simulink model "ConfiguredHevMmVirtualVehicle"  (R2025b)
settings: configuration reference "VehicleVariable" (kept outside this file)
StartFcn:
  | %tic
StopFcn:
  | %toc
model workspace (MAT data in the model file):
  ExtDrvCmdsSwitch : Simulink.Parameter (value not decoded)
  ExtDrvRefSwitch : Simulink.Parameter (value not decoded)
  ExtEnvSwitch : Simulink.Parameter (value not decoded)
  ExtGndSwitch : Simulink.Parameter (value not decoded)
symbols that are objects in the model workspace (value not decoded): ExtDrvCmdsSwitch, ExtDrvRefSwitch, ExtEnvSwitch, ExtGndSwitch
undefined symbols (not defined in the file or in its folder): AmbTemp, BaroPress, CurvGradRef, CurvRef, DCM, DriverAeroRes, DriverDrivelineRes, DriverInitialGear, DriverPreviewDist, DriverRollRes, DriverShiftTime, DriverTimeConst, DriverTractiveForce, EnvAbsPrs, EnvAirTemp, EnvGrvty, EnvNomFrictionScaling, EnvNominalGrade, EnvScnFrictionMap, EnvScnFrictionMapXBpts, EnvScnFrictionMapYBpts, EnvScnHeightMap, EnvScnHeightMapXBpts, EnvScnHeightMapYBpts, EnvWindVelX, EnvWindVelY, EnvWindVelZ, Gnd, Grade, HazzardCmd, HighBeamCmd, lambda_mux, LeftSignalCmd, LngRef, LowBeamCmd, LtrRef, PhiRef, PlntVehDstCGFrntAxl, PlntVehDstCGRearAxl, PlntVehInitLatPos, PlntVehInitLongPos, PlntVehInitPitchAng, PlntVehInitRollAng, PlntVehInitVertPos, PlntVehInitYawAng, PlntVehMass, PlntVehTrckWdth, PlntVehYawMomentInertia, PlntWhlLdRadiusFrnt, PlntWhlLdRadiusRear, RightSignalCmd, ScnCRRadius, Sim3dSensor, Wind, XRef, YRef, Z
libraries: simulink x28, autolibutils x8, autolibsharedcommon x7, vehdynlibscenariocommon x7, vehdynlibviscommon x4, vehdynlibdriver x2, sim3dgroundtruthsensorlib x2, sim3dlib x2, autolibshared x2, sim3dautolib x2, sl3dlib x1, sharedtransform x1
(part 6 of 6)

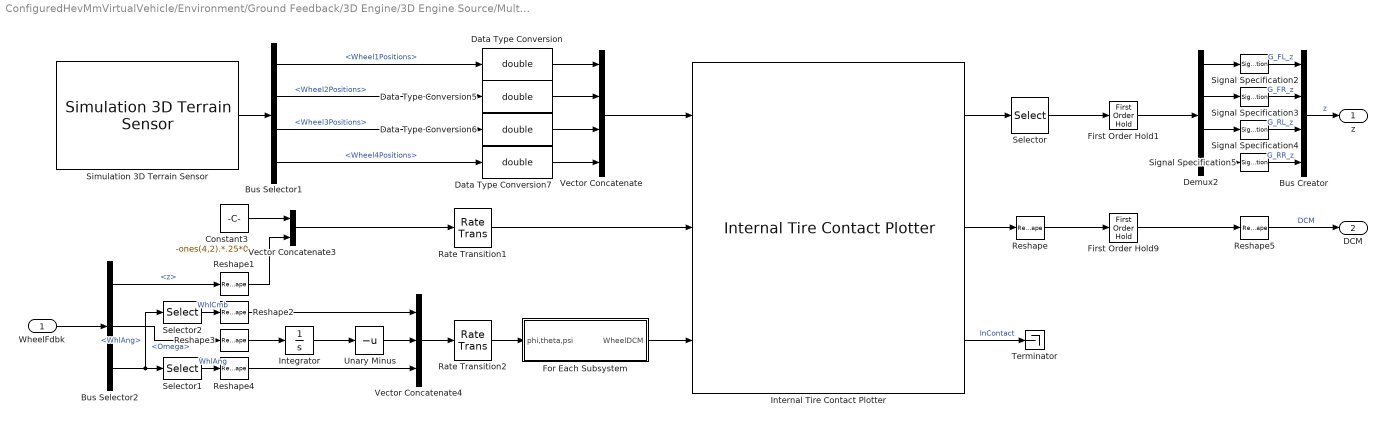
== system ConfiguredHevMmVirtualVehicle/Environment/Ground Feedback/3D Engine/3D Engine Source/Multiple Points ==
  WheelFdbk : Inport
  Bus Creator : BusCreator  Inputs=4
  Bus Selector1 : BusSelector  OutputSignals=Wheel1Positions,Wheel2Positions,Wheel3Positions,Wheel4Positions
  Bus Selector2 : BusSelector  OutputSignals=z,Omega,WhlAng
  Constant3 : Constant  Value=-ones(4,2).*.25*0
  Data Type Conversion{,5..7} (4 alike) : DataTypeConversion  OutDataTypeStr=double  SaturateOnIntegerOverflow=off  RndMeth=Floor
  Demux2 : Demux
  First Order Hold1 : FirstOrderHold  OutputAlgorithm=Fast (Minimize Error)  ErrorTolerance=.001
  First Order Hold9 : FirstOrderHold  InitialOutput=reshape(repmat(eye(3),1,1,4),[],1)  OutputAlgorithm=Fast (Minimize Error)  ErrorTolerance=.001
  For Each Subsystem : Subsystem  TreatAsAtomicUnit=on
  Integrator : Integrator  WrapState=on  ZeroCross=off
  Internal Tire Contact Plotter : vehdynlibviscommon/Internal Tire Contact Plotter  dispFig=off  numAxles=2  numWheelsPerAxle=2  wheelRad=.33  wheelWidth=.235  rayOrigins=[0.5 -0.5 0;0.4 -0.5 0;0.3 -0.5 0;0.19999999999999996 -0.5 0;0.099999999999999978 -0.5 0;0 -0.5 0;-0.099999999999999978 -0.5 0;-0.19999999999999996 -0.5 0;-0.3 -0.5 0;-0.4 -0.5 0;-0.5 -0.5 0;0.5 -0.4 0;0.4 -0.4 0;0.3 -0.4 0;0.19999999999999996 -0.4 0;0.099999999999999978 -0.4 0;0 -0.4 0;-0.099999999999999978 -0.4 0;-0.19999999999999996 -0.4 0;-0.3 -0.4 0;-0.4 -0.4 0;-0.5 -0.4 0;0.5 -0.3 0;0.4 -0.3 0;0.3 -0.3 0;0.19999999999999996 -0.3 0;0.099999999999999978 -0.3 0;0 -0.3 0;-0.099999999999999978 -0.3 0;-0.19999999999999996 -0.3 0;-0.3 -0.3 0;-0.4 -0.3 0;-0.5 -0.3 0;0.5 -0.19999999999999996 0;0.4 -0.19999999999999996 0;0.3 -0.19999999999999996 0;0.19999999999999996 -0.19999999999999996 0;0.099999999999999978 -0.19999999999999996 0;0 -0.19999999999999996 0;-0.099999999999999978 -0.19999999999999996 0;-0.19999999999999996 -0.19999999999999996 0;-0.3 -0.19999999999999996 0;-0.4 -0.19999999999999996 0;-0.5 -0.19999999999999996 0;0.5 -0.099999999999999978 0;0.4 -0.099999999999999978 0;0.3 -0.099999999999999978 0;0.19999999999999996 -0.099999999999999978 0;0.099999999999999978 -0.099999999999999978 0;0 -0.099999999999999978 0;-0.099999999999999978 -0.099999999999999978 0;-0.19999999999999996 -0.099999999999999978 0;-0.3 -0.099999999999999978 0;-0.4 -0.099999999999999978 0;-0.5 -0.099999999999999978 0;0.5 0 0;0.4 0 0;0.3 0 0;0.19999999999999996 0 0;0.099999999999999978 0 0;0 0 0;-0.099999999999999978 0 0;-0.19999999999999996 0 0;-0.3 0 0;-0.4 0 0;-0.5 0 0;0.5 0.099999999999999978 0;0.4 0.099999999999999978 0;0.3 0.099999999999999978 0;0.19999999999999996 0.099999999999999978 0;0.099999999999999978 0.099999999999999978 0;0 0.099999999999999978 0;-0.099999999999999978 0.099999999999999978 0;-0.19999999999999996 0.099999999999999978 0;-0.3 0.099999999999999978 0;-0.4 0.099999999999999978 0;-0.5 0.099999999999999978 0;0.5 0.19999999999999996 0;0.4 0.19999999999999996 0;0.3 0.19999999999999996 0;0.19999999999999996 0.19999999999999996 0;0.099999999999999978 0.19999999999999996 0;0 0.19999999999999996 0;-0.099999999999999978 0.19999999999999996 0;-0.19999999999999996 0.19999999999999996 0;-0.3 0.19999999999999996 0;-0.4 0.19999999999999996 0;-0.5 0.19999999999999996 0;0.5 0.3 0;0.4 0.3 0;0.3 0.3 0;0.19999999999999996 0.3 0;0.099999999999999978 0.3 0;0 0.3 0;-0.099999999999999978 0.3 0;-0.19999999999999996 0.3 0;-0.3 0.3 0;-0.4 0.3 0;-0.5 0.3 0;0.5 0.4 0;0.4 0.4 0;0.3 0.4 0;0.19999999999999996 0.4 0;0.099999999999999978 0.4 0;0 0.4 0;-0.099999999999999978 0.4 0;-0.19999999999999996 0.4 0;-0.3 0.4 0;-0.4 0.4 0;-0.5 0.4 0;0.5 0.5 0;0.4 0.5 0;0.3 0.5 0;0.19999999999999996 0.5 0;0.099999999999999978 0.5 0;0 0.5 0;-0.099999999999999978 0.5 0;-0.19999999999999996 0.5 0;-0.3 0.5 0;-0.4 0.5 0;-0.5 0.5 0]
  Rate Transition1 : RateTransition  Integrity=off  Deterministic=off  OutPortSampleTime=.01
  Rate Transition2 : RateTransition  Integrity=off  Deterministic=off  OutPortSampleTime=.01
  Reshape : Reshape  OutputDimensionality=Column vector (2-D)
  Reshape1 : Reshape  OutputDimensionality=Column vector (2-D)
  Reshape2 : Reshape  OutputDimensionality=Row vector (2-D)
  Reshape3 : Reshape  OutputDimensionality=Row vector (2-D)
  Reshape4 : Reshape  OutputDimensionality=Row vector (2-D)
  Reshape5 : Reshape  OutputDimensionality=Customize  OutputDimensions=[3,3,4]
  Selector : Selector  NumberOfDimensions=2  InputPortWidth=3  IndexOptions=Select all,Index vector (dialog)  Indices=[1 3],3  OutputSizes=1,1
  Selector1 : Selector  NumberOfDimensions=2  InputPortWidth=3  IndexOptions=Index vector (dialog),Select all  Indices=[3],1  OutputSizes=1,1
  Selector2 : Selector  NumberOfDimensions=2  InputPortWidth=3  IndexOptions=Index vector (dialog),Select all  Indices=[1],1  OutputSizes=1,1
  Signal Specification{2..5} (4 alike) : SignalSpecification  Unit=m
  Simulation 3D Terrain Sensor : sim3dgroundtruthsensorlib/Simulation 3D Terrain Sensor  Priority=1  vehTagList={'Scene Origin';'SimulinkVehicle1';'0'}  sensorTag=Sim3dSensor�  sensorId=1  sensorName=Sim3dSensor�  vehTag=SimulinkVehicle1  CoordinateSystem=Default  tmountOffset=[0, 0, 0]  rmountOffset=[0,0,0,]  RayOrigins=[0.5 -0.5 0;0.4 -0.5 0;0.3 -0.5 0;0.19999999999999996 -0.5 0;0.099999999999999978 -0.5 0;0 -0.5 0;-0.099999999999999978 -0.5 0;-0.19999999999999996 -0.5 0;-0.3 -0.5 0;-0.4 -0.5 0;-0.5 -0.5 0;0.5 -0.4 0;0.4 -0.4 0;0.3 -0.4 0;0.19999999999999996 -0.4 0;0.099999999999999978 -0.4 0;0 -0.4 0;-0.099999999999999978 -0.4 0;-0.19999999999999996 -0.4 0;-0.3 -0.4 0;-0.4 -0.4 0;-0.5 -0.4 0;0.5 -0.3 0;0.4 -0.3 0;0.3 -0.3 0;0.19999999999999996 -0.3 0;0.099999999999999978 -0.3 0;0 -0.3 0;-0.099999999999999978 -0.3 0;-0.19999999999999996 -0.3 0;-0.3 -0.3 0;-0.4 -0.3 0;-0.5 -0.3 0;0.5 -0.19999999999999996 0;0.4 -0.19999999999999996 0;0.3 -0.19999999999999996 0;0.19999999999999996 -0.19999999999999996 0;0.099999999999999978 -0.19999999999999996 0;0 -0.19999999999999996 0;-0.099999999999999978 -0.19999999999999996 0;-0.19999999999999996 -0.19999999999999996 0;-0.3 -0.19999999999999996 0;-0.4 -0.19999999999999996 0;-0.5 -0.19999999999999996 0;0.5 -0.099999999999999978 0;0.4 -0.099999999999999978 0;0.3 -0.099999999999999978 0;0.19999999999999996 -0.099999999999999978 0;0.099999999999999978 -0.099999999999999978 0;0 -0.099999999999999978 0;-0.099999999999999978 -0.099999999999999978 0;-0.19999999999999996 -0.099999999999999978 0;-0.3 -0.099999999999999978 0;-0.4 -0.099999999999999978 0;-0.5 -0.099999999999999978 0;0.5 0 0;0.4 0 0;0.3 0 0;0.19999999999999996 0 0;0.099999999999999978 0 0;0 0 0;-0.099999999999999978 0 0;-0.19999999999999996 0 0;-0.3 0 0;-0.4 0 0;-0.5 0 0;0.5 0.099999999999999978 0;0.4 0.099999999999999978 0;0.3 0.099999999999999978 0;0.19999999999999996 0.099999999999999978 0;0.099999999999999978 0.099999999999999978 0;0 0.099999999999999978 0;-0.099999999999999978 0.099999999999999978 0;-0.19999999999999996 0.099999999999999978 0;-0.3 0.099999999999999978 0;-0.4 0.099999999999999978 0;-0.5 0.099999999999999978 0;0.5 0.19999999999999996 0;0.4 0.19999999999999996 0;0.3 0.19999999999999996 0;0.19999999999999996 0.19999999999999996 0;0.099999999999999978 0.19999999999999996 0;0 0.19999999999999996 0;-0.099999999999999978 0.19999999999999996 0;-0.19999999999999996 0.19999999999999996 0;-0.3 0.19999999999999996 0;-0.4 0.19999999999999996 0;-0.5 0.19999999999999996 0;0.5 0.3 0;0.4 0.3 0;0.3 0.3 0;0.19999999999999996 0.3 0;0.099999999999999978 0.3 0;0 0.3 0;-0.099999999999999978 0.3 0;-0.19999999999999996 0.3 0;-0.3 0.3 0;-0.4 0.3 0;-0.5 0.3 0;0.5 0.4 0;0.4 0.4 0;0.3 0.4 0;0.19999999999999996 0.4 0;0.099999999999999978 0.4 0;0 0.4 0;-0.099999999999999978 0.4 0;-0.19999999999999996 0.4 0;-0.3 0.4 0;-0.4 0.4 0;-0.5 0.4 0;0.5 0.5 0;0.4 0.5 0;0.3 0.5 0;0.19999999999999996 0.5 0;0.099999999999999978 0.5 0;0 0.5 0;-0.099999999999999978 0.5 0;-0.19999999999999996 0.5 0;-0.3 0.5 0;-0.4 0.5 0;-0.5 0.5 0]  RayDirections=[0 0 -1;0 0 -1;0 0 -1;0 0 -1;0 0 -1;0 0 -1;0 0 -1;0 0 -1;0 0 -1;0 0 -1;0 0 -1;0 0 -1;0 0 -1;0 0 -1;0 0 -1;0 0 -1;0 0 -1;0 0 -1;0 0 -1;0 0 -1;0 0 -1;0 0 -1;0 0 -1;0 0 -1;0 0 -1;0 0 -1;0 0 -1;0 0 -1;0 0 -1;0 0 -1;0 0 -1;0 0 -1;0 0 -1;0 0 -1;0 0 -1;0 0 -1;0 0 -1;0 0 -1;0 0 -1;0 0 -1;0 0 -1;0 0 -1;0 0 -1;0 0 -1;0 0 -1;0 0 -1;0 0 -1;0 0 -1;0 0 -1;0 0 -1;0 0 -1;0 0 -1;0 0 -1;0 0 -1;0 0 -1;0 0 -1;0 0 -1;0 0 -1;0 0 -1;0 0 -1;0 0 -1;0 0 -1;0 0 -1;0 0 -1;0 0 -1;0 0 -1;0 0 -1;0 0 -1;0 0 -1;0 0 -1;0 0 -1;0 0 -1;0 0 -1;0 0 -1;0 0 -1;0 0 -1;0 0 -1;0 0 -1;0 0 -1;0 0 -1;0 0 -1;0 0 -1;0 0 -1;0 0 -1;0 0 -1;0 0 -1;0 0 -1;0 0 -1;0 0 -1;0 0 -1;0 0 -1;0 0 -1;0 0 -1;0 0 -1;0 0 -1;0 0 -1;0 0 -1;0 0 -1;0 0 -1;0 0 -1;0 0 -1;0 0 -1;0 0 -1;0 0 -1;0 0 -1;0 0 -1;0 0 -1;0 0 -1;0 0 -1;0 0 -1;0 0 -1;0 0 -1;0 0 -1;0 0 -1;0 0 -1;0 0 -1;0 0 -1;0 0 -1;0 0 -1;0 0 -1;0 0 -1]  RayLengths=[20;20;20;20;20;20;20;20;20;20;20;20;20;20;20;20;20;20;20;20;20;20;20;20;20;20;20;20;20;20;20;20;20;20;20;20;20;20;20;20;20;20;20;20;20;20;20;20;20;20;20;20;20;20;20;20;20;20;20;20;20;20;20;20;20;20;20;20;20;20;20;20;20;20;20;20;20;20;20;20;20;20;20;20;20;20;20;20;20;20;20;20;20;20;20;20;20;20;20;20;20;20;20;20;20;20;20;20;20;20;20;20;20;20;20;20;20;20;20;20;20]  NumberOfWheels=4  VisualizeTraceLines=off  SampleTime=-1  aMode=2  ID=1
  Terminator : Terminator
  Unary Minus : UnaryMinus
  Vector Concatenate : Concatenate  NumInputs=4  Mode=Multidimensional array  ConcatenateDimension=3
  Vector Concatenate3 : Concatenate  Mode=Multidimensional array  ConcatenateDimension=2
  Vector Concatenate4 : Concatenate  NumInputs=3  Mode=Multidimensional array
  z : Outport
  DCM : Outport  Port=2
  wires:
  Data Type Conversion6/1 -> Vector Concatenate/3
  Selector/1 -> First Order Hold1/1
  Signal Specification5/1 -> Bus Creator/4  "G_RR_z"
  Bus Selector1/3 -> Data Type Conversion6/1  "<Wheel3Positions>"
  Demux2/2 -> Signal Specification3/1
  Data Type Conversion/1 -> Vector Concatenate/1
  Data Type Conversion5/1 -> Vector Concatenate/2
  Demux2/3 -> Signal Specification4/1
  Internal Tire Contact Plotter/1 -> Selector/1
  Internal Tire Contact Plotter/3 -> Terminator/1  "InContact"
  Vector Concatenate/1 -> Internal Tire Contact Plotter/1
  Data Type Conversion7/1 -> Vector Concatenate/4
  Bus Selector1/1 -> Data Type Conversion/1  "<Wheel1Positions>"
  Demux2/4 -> Signal Specification5/1
  Bus Creator/1 -> z/1  "z"
  Signal Specification2/1 -> Bus Creator/1  "G_FL_z"
  Bus Selector1/4 -> Data Type Conversion7/1  "<Wheel4Positions>"
  Signal Specification3/1 -> Bus Creator/2  "G_FR_z"
  Signal Specification4/1 -> Bus Creator/3  "G_RL_z"
  Bus Selector1/2 -> Data Type Conversion5/1  "<Wheel2Positions>"
  Demux2/1 -> Signal Specification2/1
  Simulation 3D Terrain Sensor/1 -> Bus Selector1/1
  Reshape5/1 -> DCM/1  "DCM"
  Internal Tire Contact Plotter/2 -> Reshape/1
  Integrator/1 -> Unary Minus/1
  Bus Selector2/2 -> Reshape3/1  "<Omega>"
  Vector Concatenate3/1 -> Rate Transition1/1
  For Each Subsystem/1(WheelDCM) -> Internal Tire Contact Plotter/3
  Reshape3/1 -> Integrator/1
  Vector Concatenate4/1 -> Rate Transition2/1
  Reshape4/1 -> Vector Concatenate4/3
  Rate Transition2/1 -> For Each Subsystem/1(phi,theta,psi)
  Reshape1/1 -> Vector Concatenate3/2
  WheelFdbk/1 -> Bus Selector2/1
  Bus Selector2/1 -> Reshape1/1  "<z>"
  Bus Selector2/3 -> Selector2/1, Selector1/1  "<WhlAng>"
  Constant3/1 -> Vector Concatenate3/1
  Reshape2/1 -> Vector Concatenate4/1
  Unary Minus/1 -> Vector Concatenate4/2
  Rate Transition1/1 -> Internal Tire Contact Plotter/2
  First Order Hold9/1 -> Reshape5/1
  Reshape/1 -> First Order Hold9/1
  First Order Hold1/1 -> Demux2/1
  Selector1/1 -> Reshape4/1  "WhlAng"
  Selector2/1 -> Reshape2/1  "WhlCmb"

== system ConfiguredHevMmVirtualVehicle/Environment/Ground Feedback/3D Engine/3D Engine Source/Single Point ==
  Bus Creator1 : BusCreator  Inputs=4
  Bus Selector2 : BusSelector  OutputSignals=Wheel1Positions,Wheel2Positions,Wheel3Positions,Wheel4Positions
  Constant2 : Constant  Value=repmat(eye(3),1,1,4)  SampleTime=-1
  Data Type Conversion{1..4} (4 alike) : DataTypeConversion  SaturateOnIntegerOverflow=off  RndMeth=Floor
  First Order Hold{5..8} (4 alike) : FirstOrderHold  ErrorTolerance=1
  Range Limiter{5..8} (4 alike) : Saturate  UpperLimit=1e3  LowerLimit=-1e3  ZeroCross=off
  Signal Specification{6..9} (4 alike) : SignalSpecification  Unit=m
  Simulation 3D Terrain Sensor1 : sim3dgroundtruthsensorlib/Simulation 3D Terrain Sensor  Priority=1  vehTagList={'Scene Origin';'SimulinkVehicle1'}  sensorTag=Sim3dSensor�  sensorId=1  sensorName=Sim3dSensor1  vehTag=SimulinkVehicle1  CoordinateSystem=Default  tmountOffset=[0, 0, 0]  rmountOffset=[0,0,0,]  RayOrigins=[0 0 1]  RayDirections=[0 0 -1]  RayLengths=20  NumberOfWheels=4  VisualizeTraceLines=off  SampleTime=-1  aMode=2  ID=1
  Zend Select{1..4} (4 alike) : Selector  NumberOfDimensions=2  InputPortWidth=3  IndexOptions=Select all,Index vector (dialog)  Indices=[1 3],3  OutputSizes=1,1
  z : Outport
  DCM : Outport  Port=2
  wires:
  Signal Specification6/1 -> Bus Creator1/1  "G_FL_z"
  Simulation 3D Terrain Sensor1/1 -> Bus Selector2/1
  Bus Selector2/4 -> Range Limiter8/1  "<Wheel4Positions>"
  Zend Select1/1 -> Data Type Conversion1/1
  Signal Specification7/1 -> Bus Creator1/2  "G_FR_z"
  Bus Selector2/2 -> Range Limiter6/1  "<Wheel2Positions>"
  Data Type Conversion3/1 -> First Order Hold7/1
  Data Type Conversion4/1 -> First Order Hold8/1
  Zend Select3/1 -> Data Type Conversion3/1
  First Order Hold6/1 -> Signal Specification7/1
  Zend Select2/1 -> Data Type Conversion2/1
  Data Type Conversion2/1 -> First Order Hold6/1
  Range Limiter6/1 -> Zend Select2/1
  Data Type Conversion1/1 -> First Order Hold5/1
  First Order Hold7/1 -> Signal Specification8/1
  Zend Select4/1 -> Data Type Conversion4/1
  Range Limiter8/1 -> Zend Select4/1
  Bus Selector2/1 -> Range Limiter5/1  "<Wheel1Positions>"
  First Order Hold8/1 -> Signal Specification9/1
  Bus Selector2/3 -> Range Limiter7/1  "<Wheel3Positions>"
  Range Limiter7/1 -> Zend Select3/1
  First Order Hold5/1 -> Signal Specification6/1
  Range Limiter5/1 -> Zend Select1/1
  Signal Specification8/1 -> Bus Creator1/3  "G_RL_z"
  Signal Specification9/1 -> Bus Creator1/4  "G_RR_z"
  Bus Creator1/1 -> z/1  "z"
  Constant2/1 -> DCM/1  "DCM"

== system ConfiguredHevMmVirtualVehicle/Environment/Ground Feedback/Ideal Inclined Plane/Ideal Inclined Plane/Enabled ==
  Z : Inport
  phi : Inport  Port=2
  theta : Inport  Port=3
  Disabled : Subsystem  VariantControl=plane3D==0
  Enabled : Subsystem  VariantControl=plane3D==1

== system ConfiguredHevMmVirtualVehicle/Environment/Subsystem/Estimated Grade/Variant Subsystem/Three-Axle ==
  Gnd : Inport
  Selector : Selector  InputPortWidth=6  IndexOptions=Index vector (dialog)  Indices=[1 2]  OutputSizes=1
  Selector1 : Selector  InputPortWidth=6  IndexOptions=Index vector (dialog)  Indices=[5 6]  OutputSizes=1
  F : Outport
  R : Outport  Port=2
  wires:
  Selector/1 -> F/1
  Gnd/1 -> Selector1/1, Selector/1
  Selector1/1 -> R/1

== system ConfiguredHevMmVirtualVehicle/Environment/Subsystem/Estimated Grade/Variant Subsystem/Two-Axle ==
  Gnd : Inport
  Selector : Selector  InputPortWidth=4  IndexOptions=Index vector (dialog)  Indices=[1 2]  OutputSizes=1
  Selector1 : Selector  InputPortWidth=4  IndexOptions=Index vector (dialog)  Indices=[3 4]  OutputSizes=1
  F : Outport
  R : Outport  Port=2
  wires:
  Selector1/1 -> R/1
  Selector/1 -> F/1
  Gnd/1 -> Selector1/1, Selector/1

== system ConfiguredHevMmVirtualVehicle/Environment/Varying Friction/Varying Friction/Road Track Friction/2D Lookup Tbl for Scaling Fctr (Lambda) ==
  XWhl : Inport  Partition=on  PartitionDimension=1  PartitionWidth=1  PartitionOffset=0
  YWhl : Inport  Port=2  Partition=on  PartitionDimension=1  PartitionWidth=1  PartitionOffset=0
  XBpt : Inport  Port=3
  YBpt : Inport  Port=4
  2-D Lookup Table : Lookup_n-D  BreakpointsForDimension1Source=Input port  BreakpointsForDimension1=xbr  BreakpointsForDimension2Source=Input port  BreakpointsForDimension2=ybr  Table=mutable  ExtrapMethod=Clip  InternalRulePriority=Speed  RndMeth=Simplest
      settings: InputPortMap=u0,u1,p5,p7
  For Each : ForEach  DisableCoverage=on
  Lambda for each whl : Outport  ConcatenationDimension=1
  wires:
  XWhl/1 -> 2-D Lookup Table/1
  YWhl/1 -> 2-D Lookup Table/2
  2-D Lookup Table/1 -> Lambda for each whl/1
  XBpt/1 -> 2-D Lookup Table/3
  YBpt/1 -> 2-D Lookup Table/4

== system ConfiguredHevMmVirtualVehicle/Environment/Varying Friction/Varying Friction/Road Track Friction/Creating Inertial Frm Bpt ==
  XCg : Inport
  YCg : Inport  Port=2
  Enable : EnablePort
  Add : Sum
  Add1 : Sum
  Constant1 : Constant  Value=ybr
  Constant3 : Constant  Value=xbr
  XBpt : Outport
  YBpt : Outport  Port=2
  wires:
  Add/1 -> XBpt/1
  Constant1/1 -> Add1/1
  Add1/1 -> YBpt/1
  Constant3/1 -> Add/2
  YCg/1 -> Add1/2
  XCg/1 -> Add/1

== system ConfiguredHevMmVirtualVehicle/Environment/Varying Friction/Varying Friction/Road Track Friction/En at t = 0 ==
  Clock1 : Clock
  Compare To Zero : simulink/Logic and Bit Operations/Compare To Zero  relop===  OutDataTypeStr=boolean
  Constant : Constant
  Constant2 : Constant  Value=0
  Switch1 : Switch  Criteria=u2 > Threshold  SaturateOnIntegerOverflow=off  InputSameDT=off
  Out1 : Outport
  wires:
  Clock1/1 -> Compare To Zero/1
  Constant2/1 -> Switch1/3
  Constant/1 -> Switch1/1
  Switch1/1 -> Out1/1
  Compare To Zero/1 -> Switch1/2

== system ConfiguredHevMmVirtualVehicle/Visualization/3D Engine/3D Engine/Scale/PartConcatenation ==
  BodyX : Inport
  BodyY : Inport  Port=2
  BodyZ : Inport  Port=3
  WheelFrontLeftX : Inport  Port=4
  WheelFrontLeftY : Inport  Port=5
  WheelFrontLeftZ : Inport  Port=6
  WheelFrontRightX : Inport  Port=7
  WheelFrontRightY : Inport  Port=8
  WheelFrontRightZ : Inport  Port=9
  WheelRearLeftX : Inport  Port=10
  WheelRearLeftY : Inport  Port=11
  WheelRearLeftZ : Inport  Port=12
  WheelRearRightX : Inport  Port=13
  WheelRearRightY : Inport  Port=14
  WheelRearRightZ : Inport  Port=15
  AllParts : Concatenate  NumInputs=5  Mode=Multidimensional array
  Body : Concatenate  NumInputs=3  Mode=Multidimensional array  ConcatenateDimension=2
  WheelFrontLeft : Concatenate  NumInputs=3  Mode=Multidimensional array  ConcatenateDimension=2
  WheelFrontRight : Concatenate  NumInputs=3  Mode=Multidimensional array  ConcatenateDimension=2
  WheelRearLeft : Concatenate  NumInputs=3  Mode=Multidimensional array  ConcatenateDimension=2
  WheelRearRight : Concatenate  NumInputs=3  Mode=Multidimensional array  ConcatenateDimension=2
  ConcatOut : Outport  VectorParamsAs1DForOutWhenUnconnected=off
  wires:
  WheelFrontRightZ/1 -> WheelFrontRight/3
  WheelRearLeftX/1 -> WheelRearLeft/1
  WheelRearRight/1 -> AllParts/5
  WheelRearLeftY/1 -> WheelRearLeft/2
  AllParts/1 -> ConcatOut/1
  WheelRearLeftZ/1 -> WheelRearLeft/3
  WheelRearRightY/1 -> WheelRearRight/2
  WheelFrontRightX/1 -> WheelFrontRight/1
  WheelFrontRightY/1 -> WheelFrontRight/2
  WheelRearRightZ/1 -> WheelRearRight/3
  WheelFrontRight/1 -> AllParts/3
  WheelRearLeft/1 -> AllParts/4
  Body/1 -> AllParts/1
  WheelRearRightX/1 -> WheelRearRight/1
  WheelFrontLeft/1 -> AllParts/2
  BodyY/1 -> Body/2
  WheelFrontLeftY/1 -> WheelFrontLeft/2
  WheelFrontLeftZ/1 -> WheelFrontLeft/3
  WheelFrontLeftX/1 -> WheelFrontLeft/1
  BodyZ/1 -> Body/3
  BodyX/1 -> Body/1

== system ConfiguredHevMmVirtualVehicle/Visualization/3D Engine/3D Engine/Trailer/No Trailer ==
  VehFdbk : Inport
  Terminator : Terminator
  wires:
  VehFdbk/1 -> Terminator/1

== system ConfiguredHevMmVirtualVehicle/Visualization/3D Engine/3D Engine/Trailer/One-Axle Trailer ==
  VehFdbk : Inport
  Simulation 3D Trailer : sim3dautolib/Simulation 3D Trailer  Priority=-1  Mesh=One-axle trailer  ActorName=SimulinkVehicle2  Translation=[PlntVehInitLongPos PlntVehInitLatPos -PlntVehInitVertPos; 0 0 0; 0 0 0]  Rotation=[PlntVehInitRollAng PlntVehInitPitchAng PlntVehInitYawAng; 0 0 0; 0 0 0]  SampleTime=-1  ActorType=SimulinkVehicle  ID=2  aMode=2  ActorTag=SimulinkVehicle2
      settings: LibrarySourceBlock=vehdynlibsim3d/Simulation 3D Trailer
  Trailer Rotation : Subsystem
  Trailer Translation : Subsystem
  wires:
  VehFdbk/1 -> Trailer Translation/1(Trailer), Trailer Rotation/1(Trailer)
  Trailer Rotation/1(Rotation) -> Simulation 3D Trailer/2
  Trailer Translation/1(Translation) -> Simulation 3D Trailer/1

== system ConfiguredHevMmVirtualVehicle/Environment/Ground Feedback/3D Engine/3D Engine Source/Multiple Points/For Each Subsystem ==
  phi,theta,psi : Inport  Partition=on  PartitionDimension=2  PartitionWidth=1  PartitionOffset=0
  For Each : ForEach  DisableCoverage=on
  Rotation Angles to Direction Cosine Matrix1 : sharedtransform/Rotation Angles to Direction Cosine Matrix  rotationOrder=YXZ  aMode=2
  Selector5 : Selector  InputPortWidth=3  IndexOptions=Index vector (dialog)  Indices=[2 1 3]  OutputSizes=1
  WheelDCM : Outport  ConcatenationDimension=3
  wires:
  Selector5/1 -> Rotation Angles to Direction Cosine Matrix1/1
  Rotation Angles to Direction Cosine Matrix1/1 -> WheelDCM/1
  phi,theta,psi/1 -> Selector5/1

== system ConfiguredHevMmVirtualVehicle/Environment/Ground Feedback/Ideal Inclined Plane/Ideal Inclined Plane/Enabled/Disabled ==

== system ConfiguredHevMmVirtualVehicle/Environment/Ground Feedback/Ideal Inclined Plane/Ideal Inclined Plane/Enabled/Enabled ==
  Z : Inport
  phi : Inport  Port=2
  theta : Inport  Port=3
  Constant1 : Constant  Value=[planeX/200, planeY/200, 1]
  Constant4 : Constant  Value=0
  Constant5 : Constant  Value=0
  Mux : Mux  Inputs=3
  Mux1 : Mux  Inputs=3
  Reshape : Reshape  OutputDimensionality=Row vector (2-D)
  Reshape1 : Reshape  OutputDimensionality=Row vector (2-D)
  Reshape2 : Reshape  OutputDimensionality=Row vector (2-D)
  Signal Specification2 : SignalSpecification  Unit=deg
  Signal Specification3 : SignalSpecification  Unit=rad
  Simulation 3D Actor : sim3dlib/Simulation 3D Actor  Priority=1  ActorName=Plane  ParentName=Scene Origin  Operation=Create at setup  InitScriptText=|  SampleTime=-1  Translation=[0 0 Z_o]  Rotation=[phi_o theta_o 0]  Scale=[planeX/200 planeY/200 1]  InputsText=|  aMode=5  ActorTag=Plane  ActorType=Sim3dActor  ID=C
      InitScriptText=|
      | planeSurface = sim3d.Actor('ActorName','BaseSurface');
      | Actor.propagate('CoordinateSystem',"ISO8855");
      | planeSurface.createShape('checker',[200,200,+0.03],[50 50]);
      | planeSurface.Color = [68 68 71]./100;
      | planeSurface.Translation = [0 0 0]; 
      | planeSurface.Shininess = 0;
      | planeSurface.Transparency = 0;
      | planeSurface.TextureMapping.Blend = 1;
      | planeSurface.TextureMapping.Roughness = .8;
      | World.add(planeSurface,Actor);
      InputsText=|
      | Plane.Translation
      | Plane.Rotation   
      | Plane.Scale
  Subtract : Sum  Inputs=+-
  Terminator : Terminator
  Unit Conversion1 : UnitConversion
  half plane thickness : Constant  Value=.015
  wires:
  Simulation 3D Actor/1 -> Terminator/1
  phi/1 -> Mux/1
  Constant5/1 -> Mux/3
  Reshape1/1 -> Simulation 3D Actor/2
  Constant4/1 -> Mux1/2, Mux1/1
  Reshape/1 -> Simulation 3D Actor/1
  Signal Specification2/1 -> Reshape1/1
  Reshape2/1 -> Simulation 3D Actor/3
  Constant1/1 -> Reshape2/1
  Z/1 -> Subtract/1
  Mux1/1 -> Reshape/1
  Subtract/1 -> Mux1/3
  half plane thickness/1 -> Subtract/2
  Unit Conversion1/1 -> Signal Specification2/1
  theta/1 -> Mux/2
  Signal Specification3/1 -> Unit Conversion1/1
  Mux/1 -> Signal Specification3/1

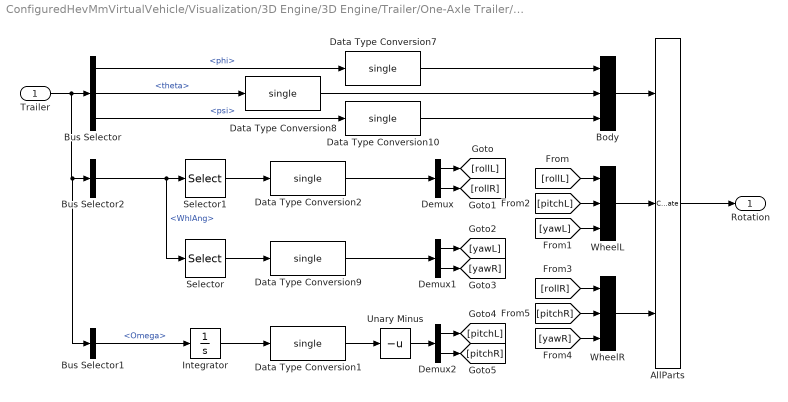
== system ConfiguredHevMmVirtualVehicle/Visualization/3D Engine/3D Engine/Trailer/One-Axle Trailer/Trailer Rotation ==
  Trailer : Inport
  AllParts : Concatenate  NumInputs=3  Mode=Multidimensional array
  Body : Concatenate  NumInputs=3  Mode=Multidimensional array  ConcatenateDimension=2
  Bus Selector : BusSelector  OutputSignals=TrlrBody.InertFrm.Cg.Ang.phi,TrlrBody.InertFrm.Cg.Ang.theta,TrlrBody.InertFrm.Cg.Ang.psi
  Bus Selector1 : BusSelector  OutputSignals=TrlrWheels.Wheels.TireFrame.Omega
  Bus Selector2 : BusSelector  OutputSignals=TrlrBody.Suspension.WhlAng
  Data Type Conversion{1..2,7..10} (6 alike) : DataTypeConversion  OutDataTypeStr=single  SaturateOnIntegerOverflow=off  RndMeth=Floor
  Demux : Demux  Outputs=2
  Demux1 : Demux  Outputs=2
  Demux2 : Demux  Outputs=2
  Integrator : Integrator  WrapState=on  WrappedStateUpperValue=2*pi  WrappedStateLowerValue=0  ZeroCross=off
  Selector : Selector  NumberOfDimensions=2  InputPortWidth=3  IndexOptions=Index vector (dialog),Select all  Indices=[3],1  OutputSizes=1,1
  Selector1 : Selector  NumberOfDimensions=2  InputPortWidth=3  IndexOptions=Index vector (dialog),Select all  Indices=[1],1  OutputSizes=1,1
  Unary Minus : UnaryMinus
  WheelL : Concatenate  NumInputs=3  Mode=Multidimensional array  ConcatenateDimension=2
  WheelR : Concatenate  NumInputs=3  Mode=Multidimensional array  ConcatenateDimension=2
  Rotation : Outport
  wires:
  Trailer/1 -> Bus Selector1/1, Bus Selector2/1, Bus Selector/1
  Body/1 -> AllParts/1
  Bus Selector/1 -> Data Type Conversion7/1  "<phi>"
  Bus Selector/3 -> Data Type Conversion10/1  "<psi>"
  Bus Selector/2 -> Data Type Conversion8/1  "<theta>"
  Selector/1 -> Data Type Conversion9/1
  Data Type Conversion9/1 -> Demux1/1
  Data Type Conversion2/1 -> Demux/1
  Selector1/1 -> Data Type Conversion2/1
  Bus Selector2/1 -> Selector1/1, Selector/1  "<WhlAng>"
  Bus Selector1/1 -> Integrator/1  "<Omega>"
  Integrator/1 -> Data Type Conversion1/1
  Unary Minus/1 -> Demux2/1
  Data Type Conversion1/1 -> Unary Minus/1
  Demux/1 -> [rollL]
  Demux/2 -> [rollR]
  Demux1/2 -> [yawR]
  Demux1/1 -> [yawL]
  Demux2/2 -> [pitchR]
  Demux2/1 -> [pitchL]
  [rollL] -> WheelL/1
  [yawL] -> WheelL/3
  [pitchL] -> WheelL/2
  [rollR] -> WheelR/1
  [yawR] -> WheelR/3
  [pitchR] -> WheelR/2
  WheelR/1 -> AllParts/3
  WheelL/1 -> AllParts/2
  AllParts/1 -> Rotation/1
  Data Type Conversion7/1 -> Body/1
  Data Type Conversion8/1 -> Body/2
  Data Type Conversion10/1 -> Body/3

== system ConfiguredHevMmVirtualVehicle/Visualization/3D Engine/3D Engine/Trailer/One-Axle Trailer/Trailer Translation ==
  Trailer : Inport
  AllParts : Concatenate  NumInputs=3  Mode=Multidimensional array
  Body : Concatenate  NumInputs=3  Mode=Multidimensional array  ConcatenateDimension=2
  Bus Selector : BusSelector  OutputSignals=TrlrBody.InertFrm.HitchF.Disp.X,TrlrBody.InertFrm.HitchF.Disp.Y,TrlrBody.InertFrm.Cg.Disp.Z
  Bus Selector1 : BusSelector  OutputSignals=TrlrBody.Suspension.dz
  Constant : Constant  Value=0  OutDataTypeStr=single
  Constant1 : Constant  Value=0  OutDataTypeStr=single
  Data Type Conversion{1,7..8,10} (4 alike) : DataTypeConversion  OutDataTypeStr=single  SaturateOnIntegerOverflow=off  RndMeth=Floor
  Demux : Demux  Outputs=2
  Unary Minus1 : UnaryMinus
  WheelL : Concatenate  NumInputs=3  Mode=Multidimensional array  ConcatenateDimension=2
  WheelR : Concatenate  NumInputs=3  Mode=Multidimensional array  ConcatenateDimension=2
  Translation : Outport
  wires:
  Trailer/1 -> Bus Selector1/1, Bus Selector/1
  Bus Selector/1 -> Data Type Conversion7/1  "<X>"
  Bus Selector/2 -> Data Type Conversion8/1  "<Y>"
  Bus Selector/3 -> Data Type Conversion10/1  "<Z>"
  Data Type Conversion7/1 -> Body/1
  Data Type Conversion8/1 -> Body/2
  Data Type Conversion10/1 -> Body/3
  Unary Minus1/1 -> Demux/1
  Bus Selector1/1 -> Data Type Conversion1/1  "<dz>"
  WheelL/1 -> AllParts/2
  Body/1 -> AllParts/1
  AllParts/1 -> Translation/1
  WheelR/1 -> AllParts/3
  Demux/1 -> [zL]
  Demux/2 -> [zR]
  [zR] -> WheelR/3
  [zL] -> WheelL/3
  Constant/1 -> WheelL/2, WheelL/1
  Constant1/1 -> WheelR/2, WheelR/1
  Data Type Conversion1/1 -> Unary Minus1/1

== matlab function ConfiguredHevMmVirtualVehicle/Environment/Ground Feedback/Ideal Inclined Plane/Ideal Inclined Plane/Z Plane ==
  data: X input; Z output; Y input; Zoffset input; phi input; theta input; DCM output
function [Z,DCM] = Zplane(X,Y,Zoffset,phi,theta)%#codege
 coder.allowpcode('plain')
 [Z,DCM] = vdynblksZplane(X,Y,Zoffset,phi,theta);
end
